simulink model "tractor_mu2018"  (R2018a)
settings: Solver=FixedStepDiscrete  StartTime=0.0  StopTime=30  FixedStep=0.001  RelTol=1e-3
model workspace (MAT data in the model file):
  MCOS : class17 (value not decoded)
undefined symbols (not defined in the file): A, a, B, b, C, D, DiscIntNeverNeededParam, Iz, K, k1, K1, k2, K2, L1, L2, m, magnitude, Phi, Sample_time, Steer_Ratio
libraries: simulink x39, Solver_SF x1, dsparch4 x1
(part 5 of 5)

== matlab function tractor_mu2018/PID_Controller//直线循迹/MATLAB Function2 ==
  data: st input; flag_ctrl output; flag_cnt output; yaw input; throttle input; yaw_ref output
function [flag_ctrl, flag_cnt, yaw_ref] = StraightModeDetector(st, yaw, throttle)

%% 实车调试版本
% 所有 persistent 变量必须为 single 以满足实车要求 
persistent ctrl_cnt yaw_sum yaw_time yaw_ref_int yaw_f
if isempty(ctrl_cnt)
    ctrl_cnt    = single(0);
    yaw_sum     = single(0);
    yaw_time    = single(0);
    yaw_ref_int = single(0);
    yaw_f       = single(0);
end

%% === 参数 ===
st_lim_enter = single(1);     % 进入判定阈值 (deg)
st_lim_exit  = single(1.2);     % 退出判定（滞回）
thr_min      = single(1);       % 油门下限 (%)
thr_max      = single(50);      % 油门上限 (%)


T_ctrl   = single(3.0);         % 需要检测的直行时间 (s)
Ts       = single(0.02);        % sample time
num_ctrl = single(T_ctrl / Ts); % 循环次数

alpha = single(0.15);           % LPF 低通滤波器系数
flag_cnt = single(0);           % 累加计算目标航向使能

%% === Step 1: LPF 过滤 yaw ===
yaw_f = yaw_f + alpha * (yaw - yaw_f);

%% === Step 2: 判断是否满足直行条件 ===
cond_enter = (abs(st) < st_lim_enter) && (throttle > thr_min) && (throttle < thr_max);
cond_exit  = (abs(st) > st_lim_exit)  || (throttle <= thr_min) || (throttle >= thr_max);

%% === Step 3: 计数器逻辑 ===
if cond_enter
    ctrl_cnt = ctrl_cnt + 1;
else
    ctrl_cnt = single(0);
end

%% === Step 4: yaw 采样（累加）===
if cond_enter && (ctrl_cnt <= num_ctrl)
    yaw_sum  = yaw_sum  + yaw_f;
    yaw_time = yaw_time + 1;
    flag_cnt = single(1);
end

%% === Step 5: 进入直线控制模式的瞬间冻结 yaw_ref ===
% if ctrl_cnt == num_ctrl
%     yaw_ref_int = yaw_sum / yaw_time;
% end
if (ctrl_cnt >= num_ctrl) && (yaw_time > 0) && (yaw_ref_int == 0)
    yaw_ref_int = yaw_sum / yaw_time;
end

%% === Step 6: 若退出模式，则清空状态 ===
if cond_exit
    ctrl_cnt    = single(0);
    yaw_sum     = single(0);
    yaw_time    = single(0);
    yaw_ref_int = single(0);
end

%% === Step 7: 输出 ===
flag_ctrl = single(ctrl_cnt >= num_ctrl);
yaw_ref   = yaw_ref_int;

end

== matlab function tractor_mu2018/PID_Controller//直线循迹/指数加权移动平均 ==
  data: uk input; y output; is_biased input

function y = ExpMovAvg(uk, is_biased)
% 指数加权移动平均滤波器
% 输入:
%   uk      : 当前输入值
%   is_biased: 是否应用偏差修正 (1=是, 0=否)
% 输出:
%   y       : 指数加权移动平均值

% 持久变量保持状态 (在时间步之间保留值)
persistent shadow count first_time decay

% 初始化参数和状态
if isempty(first_time)
    % 初始化标志
    first_time = true;
    
    % 初始化状态值
    shadow = double(0);
    count = 0;
    
    % 设置衰减因子 (0.9是常用值，可根据需要修改)
    decay = 0.9;
end

% 主处理逻辑
if first_time
    % 第一次调用 - 初始化状态
    shadow = double(uk);
    count = 1;
    first_time = false;
    y = uk;  % 第一次返回当前值
else
    % 更新计数器
    count = count + 1;
    
    % 计算指数加权平均值
     a = decay * shadow + (1 - decay) * uk;
    shadow = double(a);
    
    if is_biased
        % 应用偏差修正 (1 - decay^count)
        bias_correction = 1 - decay^count;
         b = shadow / bias_correction;
        y = single(b);
    else
        % 返回原始加权平均值
        y = single(shadow);
    end
end
end

== matlab function tractor_mu2018/PID_Controller//直线循迹/模式判断 ==
  data: v input; st input; avg input; mode output
function mode  = stateflow(v,st,avg)

mode = 7; %常规模式

% 沥青路面判断
    if avg <= 2
        if v > 20
            if st>=8
                mode = 1; % 高速转向
            elseif st<=3
                mode = 2; % 高速直行
            end
        elseif v < 10
            if st>=5
                mode = 3; % 低速转向
            elseif st<5
                mode = 4; % 低速直行
            end
        end
    % 土地路面判断
    elseif avg >= 3
        if v >= 10
            mode = 5; % 土地快速
        elseif v < 10
            mode = 6; % 土地低速
        end
    end
end
